simulink model "sschdlexVoltageSourceInverterModel"  (R2026a)
settings: Solver=FixedStepDiscrete  StopTime=0.03
InitFcn:
  | ts = 1e-005;
undefined symbols (not defined in the file or in its folder): Down, Up
libraries: fl_lib x11, nesl_utility x11, ee_lib x6, simulink x3, eeGeneralControl x1
CloseFcn:
  | clear all;
settings Model: DataTypeOverride=Off  Creator=The MathWorks, Inc.  LastModifiedBy=The MathWorks, Inc.
settings OptimizationCC: ConditionallyExecuteInputs=off
settings DebuggingCC: AlgebraicLoopMsg=error  SingleTaskRateTransMsg=error
settings HardwareCC: ProdHWDeviceType=ASIC/FPGA->ASIC/FPGA  TargetBitPerLong=64.0  TargetBitPerPointer=64.0  TargetBitPerSizeT=64.0  TargetBitPerPtrDiffT=64.0  TargetLongLongMode=on  TargetIntDivRoundTo=Zero  TargetEndianess=LittleEndian  TargetWordSize=64.0  TargetHWDeviceType=Custom Processor->MATLAB Host Computer  ProdEqTarget=off
settings SimscapeCC: SimscapeNominalValues="[{\"value\":\"1\",\"unit\":\"A\"},{\"value\":\"1\",\"unit\":\"bar\"},{\"value\":\"1\",\"unit\":\"cm^2\"},{\"value\":\"1\",\"unit\":\"cm^3/s\"},{\"value\":\"1\",\"unit\":\"kJ/kg\"},{\"value\":\"1\",\"unit\":\"kW\"},{\"value\":\"1\",\"unit\":\"l\"},{\"value\":\"1\",\"unit\":\"N\"},{\"value\":\"1\",\"unit\":\"N*m\"},{\"value\":\"1\",\"unit\":\"V\"}]"  SimscapeLogType=none  SimscapeLogDataHistory=5000.0

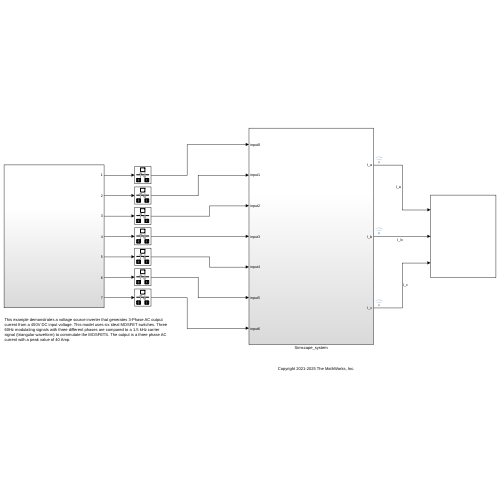
[thumbnail: Simulink's stored preview of the top-level diagram]
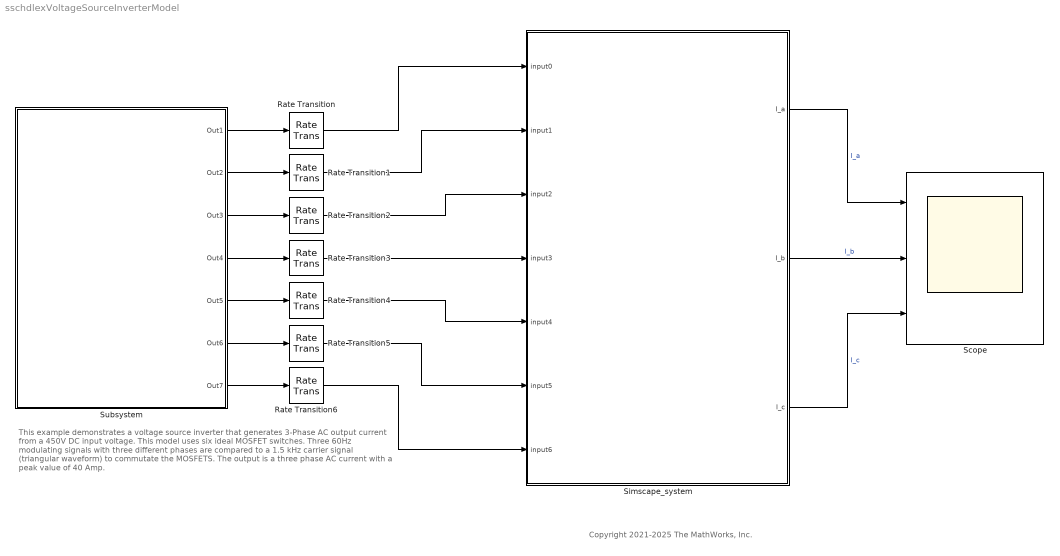
== system sschdlexVoltageSourceInverterModel ==
  note: This example demonstrates a voltage source inverter that generates 3-Phase AC output current from a 450V DC input voltage. This model uses six ideal MOSFET switches. Three 60Hz modulating signals with three different phases are compared to a 1.5 kHz carrier signal (triangular waveform) to commutate the MOSFETS. The output is a three phase AC current with a peak value of 40 Amp.
  note: Copyright 2021-2025 The MathWorks, Inc.
  Rate Transition{,1..6} (7 alike) : RateTransition
  Scope : Scope  NumInputPorts=3
      settings: ActiveDisplayYMinimum=-48.27085  ActiveDisplayYMaximum=49.00639
  Simscape_system : Subsystem
  Subsystem : Subsystem
  wires:
  Subsystem/1(Out1) -> Rate Transition/1
  Subsystem/7(Out7) -> Rate Transition6/1
  Subsystem/6(Out6) -> Rate Transition5/1
  Subsystem/5(Out5) -> Rate Transition4/1
  Subsystem/4(Out4) -> Rate Transition3/1
  Subsystem/3(Out3) -> Rate Transition2/1
  Subsystem/2(Out2) -> Rate Transition1/1
  Rate Transition/1 -> Simscape_system/1(input0)
  Rate Transition1/1 -> Simscape_system/2(input1)
  Rate Transition2/1 -> Simscape_system/3(input2)
  Rate Transition3/1 -> Simscape_system/4(input3)
  Rate Transition4/1 -> Simscape_system/5(input4)
  Rate Transition5/1 -> Simscape_system/6(input5)
  Rate Transition6/1 -> Simscape_system/7(input6)
  Simscape_system/2(I_b) -> Scope/2  "I_b"
  Simscape_system/1(I_a) -> Scope/1  "I_a"
  Simscape_system/3(I_c) -> Scope/3  "I_c"

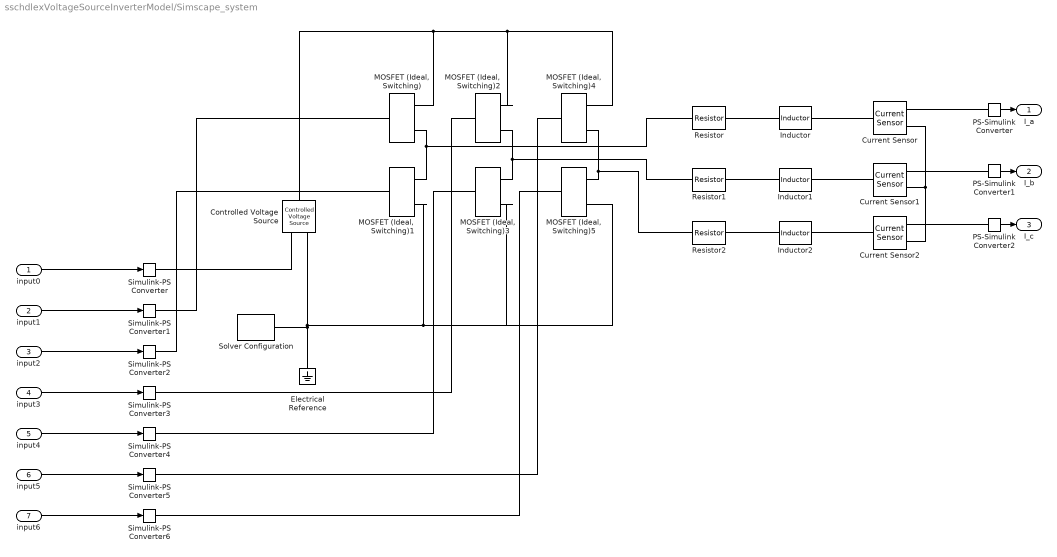
== system sschdlexVoltageSourceInverterModel/Simscape_system ==
  input0 : Inport
  input1 : Inport  Port=2
  input2 : Inport  Port=3
  input3 : Inport  Port=4
  input4 : Inport  Port=5
  input5 : Inport  Port=6
  input6 : Inport  Port=7
  Controlled Voltage Source : fl_lib/Electrical/Electrical Sources/Controlled Voltage Source
  Current Sensor : fl_lib/Electrical/Electrical Sensors/Current Sensor
  Current Sensor1 : fl_lib/Electrical/Electrical Sensors/Current Sensor
  Current Sensor2 : fl_lib/Electrical/Electrical Sensors/Current Sensor
  Electrical Reference : fl_lib/Electrical/Electrical Elements/Electrical Reference
  Inductor : fl_lib/Electrical/Electrical Elements/Inductor  l=0.0077 H  r=0 Ohm  g=1e-9 1/Ohm  i_specify=off  i_priority=None  i=0 A  i_nominal_specify=off  i_nominal_value=1  i_nominal_unit=A  v_specify=off  v_priority=None  v=0 V  v_nominal_specify=off  v_nominal_value=1  v_nominal_unit=V  i_L_specify=off  i_L_priority=High  i_L=0 A  i_L_nominal_specify=off  i_L_nominal_value=1  i_L_nominal_unit=A
  Inductor1 : fl_lib/Electrical/Electrical Elements/Inductor  l=0.0077 H  r=0 Ohm  g=1e-9 1/Ohm  i_specify=off  i_priority=None  i=0 A  i_nominal_specify=off  i_nominal_value=1  i_nominal_unit=A  v_specify=off  v_priority=None  v=0 V  v_nominal_specify=off  v_nominal_value=1  v_nominal_unit=V  i_L_specify=off  i_L_priority=High  i_L=0 A  i_L_nominal_specify=off  i_L_nominal_value=1  i_L_nominal_unit=A
  Inductor2 : fl_lib/Electrical/Electrical Elements/Inductor  l=0.0077 H  r=0 Ohm  g=1e-9 1/Ohm  i_specify=off  i_priority=None  i=0 A  i_nominal_specify=off  i_nominal_value=1  i_nominal_unit=A  v_specify=off  v_priority=None  v=0 V  v_nominal_specify=off  v_nominal_value=1  v_nominal_unit=V  i_L_specify=off  i_L_priority=High  i_L=0 A  i_L_nominal_specify=off  i_L_nominal_value=1  i_L_nominal_unit=A
  MOSFET (Ideal, Switching){,1..5} (6 alike) : ee_lib/Semiconductors & Converters/MOSFET (Ideal, Switching)  port_option=ee.enum.controlport.ps  Rds=0.001 Ohm  Goff=1e-6 1/Ohm  Vth=0.5 V  diode_param=2  diode_Vf=0.8 V  diode_Ron=0.001 Ohm  diode_Goff=1e-5 1/Ohm  diode_C=50e-9 F  diode_iRM=-235 A  diode_iF=300 A  diode_idot=-50 A/us  diode_trr_param=1  diode_trr_factor=3  diode_trr=15 us  diode_Qrr=1500 s*uA  ids_specify=off  ids_priority=None  ids=0 A  ids_nominal_specify=off  ids_nominal_value=1  ids_nominal_unit=A  vds_specify=off  vds_priority=None  vds=0 V  vds_nominal_specify=off  vds_nominal_value=1  vds_nominal_unit=V  vgs_specify=off  vgs_priority=None  vgs=0 V  vgs_nominal_specify=off  vgs_nominal_value=1  vgs_nominal_unit=V  thermal_loss_option=ee.enum.converters.thermalLossOption.constantvalues  Von_data=[0, 1.8, 3.2, 6, 10, 16; 0, 2, 5.5, 9.5, 15, 25] V  Tj=[298.15, 448.15] K  Iout_data=[0, 20, 40, 60, 80, 100] A  tabulateWithVds=false  Eon_data=[0, 55.04, 124.57, 235.53, 362.12; 0, 71.25, 161.25, 304.88, 468.75] * 1e-6 J  Eoff_data=[0, 18, 30, 56.1, 76.5; 0, 22.5, 37.5, 70.13, 95.63] * 1e-6 J  Eon_data_3D=[zeros(2, 5, 3)] J  Eoff_data_3D=[zeros(2, 5, 3)] J  Tj_loss=[298.15, 448.15] K  Iout_data_loss=[0, 10, 20, 30, 40] A  Vds_loss=[0, 150, 300] V  Eon_scalar=22.86e-3 J  Eoff_scalar=17.14e-3 J  Voff=300 V  Iout_scalar=600 A  useCurrentFromPreviousCycle=false  useVoltageFromPreviousCycle=false  diodeModelType=ee.enum.converters.diodeModelType.pwl  diodeTableType=ee.enum.diode.tableType.IfMat  diode_ReverseIVType=ee.enum.diode.diodeReverseIV.constant  diode_IfMat=[.07, .12, .19, 1.75, 4.24, 7.32, 11.2; .16, .3, .72, 2.14, 4.02, 6.35, 9.12] A  diode_VfMat=[.9, 1.15, 1.25, 1.5, 1.75, 2.17, 2.6, 2.85; .58, .68, .75, 1.1, 1.38, 1.77, 2.27, 2.7] V  diode_TjVec=[25, 125] degC  diode_VfVec=[.5, .7, .9, 1.3, 1.7, 2.1, 2.5] V  diode_IfVec=[.1, .2, .5, 1, 2, 4, 7, 10] A  diode_IrMat=[1e-06, 2e-06, 5e-06, 1e-05, 2.5e-05, 5e-05, .0001; 2e-06, 5e-06, 1e-05, 4e-05, 8e-05, .0002, .0005] A  diode_VrMat=[10, 100, 200, 250, 300, 325, 350; 10, 70, 160, 220, 270, 300, 320] V  diode_VrVec=[10, 20, 40, 50, 70, 80, 100] V  diode_IrVec=[1e-06, 2e-06, 5e-06, 1e-05, 2e-05, 5e-05, .0001] A  diode_Vr=-600 V  diode_Ls=150 nH  diode_Erec=0.03 J  diode_rec_loss_model=ee.enum.diode.reverseRecoveryModel.fixed  diode_ErecVal=0 J  diode_scaleWithIandV=true  diode_ErecMat=zeros(2, 3) J  diodeErecMat3D=zeros(2, 3, 2) J  diode_TjrecVec=[298.15, 398.15] K  diode_IfrecVec=[.1, 1, 10] A  diodeVrecVec=[0, 100] V  diode_IrecVal=10 A  diode_VrecVal=10 V  diode_tFilter=1 / 1000 / 100 s  separateThermalPortForDiode=false  thermal_network_parameterization=ee.enum.thermalNetworkTopology.external  Rth=[.03, .2] K/W  Rth_Cauer=[.03, .1, .2] K/W  Rth_Foster=[.03, .2] K/W  thermal_mass_parameterization=ee.enum.thermalNetwork.timeconstant  thermal_mass=[3, 25] J/K  thermal_mass_Cauer=[3, 10, 25] J/K  thermal_mass_Foster=[33, 50] J/K  thermal_time_constant=[.1, 5] s  thermal_time_constant_Cauer=[.1, 1, 5] s  thermal_time_constant_Foster=[1, 10] s  thermal_mass_initial_temperatures=[25, 25] degC  thermal_mass_initial_temperatures_Cauer=[25, 25, 25] degC  junction_thermal_mass=0.1 J/K  Tvec_initial_Foster=[25, 25, 25, 25] degC  RthDiode=[.03, .2] K/W  RthCauerDiode=[.03, .1, .2] K/W  RthFosterDiode=[.03, .2] K/W  thermalMassDiode=[3, 25] J/K  thermalMassCauerDiode=[3, 10, 25] J/K  thermalMassFosterDiode=[33, 50] J/K  thermalTauDiode=[.1, 5] s  thermalTauCauerDiode=[.1, 1, 5] s  thermalTauFosterDiode=[1, 10] s  thermalMassInitTempDiode=[25, 25] degC  thermalMassInitTempCauerDiode=[25, 25, 25] degC  junctionthermalMassDiode=0.1 J/K  TVecInitialFosterDiode=[25, 25, 25, 25] degC  no_thermal_network=0  mosfet_junction_temperature_specify=off  mosfet_junction_temperature_priority=None  mosfet_junction_temperature=25 degC  mosfet_junction_temperature_nominal_specify=off  mosfet_junction_temperature_nominal_value=1  mosfet_junction_temperature_nominal_unit=degC  diode_junction_temperature_specify=off  diode_junction_temperature_priority=None  diode_junction_temperature=25 degC  diode_junction_temperature_nominal_specify=off  diode_junction_temperature_nominal_value=1  diode_junction_temperature_nominal_unit=degC  Qj_specify=off  Qj_priority=None  Qj=0 W  Qj_nominal_specify=off  Qj_nominal_value=1  Qj_nominal_unit=W  accumulatedSwitchingLosses_specify=off  accumulatedSwitchingLosses_priority=None  accumulatedSwitchingLosses=0 J
  PS-Simulink Converter : nesl_utility/PS-Simulink Converter  PhysicalDomain=network_engine_domain  SubClassName=ps_output  LeftPortType=input  RightPortType=output  PseudoPeriodic=off  Frequencies=[]  VectorFormat=1-D array  Unit=inherit  AffineConversion=off
  PS-Simulink Converter1 : nesl_utility/PS-Simulink Converter  PhysicalDomain=network_engine_domain  SubClassName=ps_output  LeftPortType=input  RightPortType=output  PseudoPeriodic=off  Frequencies=[]  VectorFormat=1-D array  Unit=inherit  AffineConversion=off
  PS-Simulink Converter2 : nesl_utility/PS-Simulink Converter  PhysicalDomain=network_engine_domain  SubClassName=ps_output  LeftPortType=input  RightPortType=output  PseudoPeriodic=off  Frequencies=[]  VectorFormat=1-D array  Unit=inherit  AffineConversion=off
  Resistor : fl_lib/Electrical/Electrical Elements/Resistor  R=3.87 Ohm  i_specify=off  i_priority=None  i=0 A  i_nominal_specify=off  i_nominal_value=1  i_nominal_unit=A  v_specify=off  v_priority=None  v=0 V  v_nominal_specify=off  v_nominal_value=1  v_nominal_unit=V
  Resistor1 : fl_lib/Electrical/Electrical Elements/Resistor  R=3.87 Ohm  i_specify=off  i_priority=None  i=0 A  i_nominal_specify=off  i_nominal_value=1  i_nominal_unit=A  v_specify=off  v_priority=None  v=0 V  v_nominal_specify=off  v_nominal_value=1  v_nominal_unit=V
  Resistor2 : fl_lib/Electrical/Electrical Elements/Resistor  R=3.87 Ohm  i_specify=off  i_priority=None  i=0 A  i_nominal_specify=off  i_nominal_value=1  i_nominal_unit=A  v_specify=off  v_priority=None  v=0 V  v_nominal_specify=off  v_nominal_value=1  v_nominal_unit=V
  Simulink-PS Converter{,1..6} (7 alike) : nesl_utility/Simulink-PS Converter  PhysicalDomain=network_engine_domain  SubClassName=ps_input  LeftPortType=input  RightPortType=output  PseudoPeriodic=off  Frequencies=[]  NoiseDistribution=none  NoiseParameters=[]  Unit=1  AffineConversion=off  FilteringAndDerivatives=provide  SimscapeFilterOrder=1  InputFilterTimeConstant=0.001  UdotUserProvided=0
  Solver Configuration : nesl_utility/Solver Configuration  PhysicalDomain=network_engine_domain  SubClassName=solver  LeftPortType=input  RightPortType=generic  Tones=[]  Harmonics=[]  SimulateNoise=off  Profile=off  UseLocalSampling=off  EnableSwitchedLinearOptims=on  FrequencyDomain=off  UseCCode=off  RelTol=0.001  AbsTol=1e-06  MinStep=1e-09  ToWorkspace=off  RevertToSquareIcSolve=off  NumHomotopyIterations=100  PhasorMode=off  PhasorModeNumHarmonics=1  ConsistencySolver=NEWTON_FTOL  CanonicalOrdering=UNORDERED  OptimizeIntermediates=UNOPTIMIZED  IndexReductionMethod=DerivativeReplacement  DoDC=off  ResidualTolerance=1e-09  ConsistencyTolSource=GLOBAL  ConsistencyAbsTol=0.001  ConsistencyRelTol=0.001  ConsistencyTolFactor=0.001  UseLocalSolver=on  LocalSolverChoice=NE_BACKWARD_EULER_ADVANCER  ResolveIndetEquations=on  FunctionEvalNumThread=1  LocalSolverSampleTime=ts  DoFixedCost=off  MaxNonlinIter=1  MaxModeIter=2  ComputeImpulses=off  ImpulseIterations=1  LinearAlgebra=auto  LinearAlgebraNumThread=0  EquationFormulation=NE_TIME_EF  DelaysMemoryBudget=1024  AutomaticFiltering=on  FilteringTimeConstant=0.001  PartitionStorageMethod=AS_NEEDED  PartitionMemoryBudget=1024  PartitionMethod=ROBUST  MultibodyUseLocalSolver=off  MultibodyLocalSolverChoice=ODE1  MultibodyLocalSolverSampleTime=0.001
  I_a : Outport
  I_b : Outport  Port=2
  I_c : Outport  Port=3
  wires:
  PS-Simulink Converter2/1 -> I_c/1
  input6/1 -> Simulink-PS Converter6/1
  input2/1 -> Simulink-PS Converter2/1
  input4/1 -> Simulink-PS Converter4/1
  input5/1 -> Simulink-PS Converter5/1
  PS-Simulink Converter/1 -> I_a/1
  input3/1 -> Simulink-PS Converter3/1
  input1/1 -> Simulink-PS Converter1/1
  input0/1 -> Simulink-PS Converter/1
  PS-Simulink Converter1/1 -> I_b/1
  connections:
  Simulink-PS Converter5/RConn1 -- "MOSFET (Ideal, Switching)4"/LConn1
  Simulink-PS Converter2/RConn1 -- "MOSFET (Ideal, Switching)1"/LConn1
  Inductor1/LConn1 -- Resistor1/RConn1
  PS-Simulink Converter/LConn1 -- Current Sensor/RConn1
  Current Sensor2/LConn1 -- Inductor2/RConn1
  "MOSFET (Ideal, Switching)2"/RConn2 -- Resistor1/LConn1 -- "MOSFET (Ideal, Switching)3"/RConn1
  Inductor/LConn1 -- Resistor/RConn1
  PS-Simulink Converter2/LConn1 -- Current Sensor2/RConn1
  PS-Simulink Converter1/LConn1 -- Current Sensor1/RConn1
  "MOSFET (Ideal, Switching)4"/RConn1 -- "MOSFET (Ideal, Switching)2"/RConn1 -- Controlled Voltage Source/LConn1 -- "MOSFET (Ideal, Switching)"/RConn1
  Simulink-PS Converter3/RConn1 -- "MOSFET (Ideal, Switching)2"/LConn1
  Simulink-PS Converter/RConn1 -- Controlled Voltage Source/RConn1
  Inductor2/LConn1 -- Resistor2/RConn1
  Simulink-PS Converter6/RConn1 -- "MOSFET (Ideal, Switching)5"/LConn1
  Electrical Reference/LConn1 -- "MOSFET (Ideal, Switching)3"/RConn2 -- "MOSFET (Ideal, Switching)5"/RConn2 -- "MOSFET (Ideal, Switching)1"/RConn2 -- Controlled Voltage Source/RConn2 -- Solver Configuration/RConn1
  Current Sensor/LConn1 -- Inductor/RConn1
  "MOSFET (Ideal, Switching)4"/RConn2 -- "MOSFET (Ideal, Switching)5"/RConn1 -- Resistor2/LConn1
  Current Sensor/RConn2 -- Current Sensor1/RConn2 -- Current Sensor2/RConn2
  "MOSFET (Ideal, Switching)"/RConn2 -- Resistor/LConn1 -- "MOSFET (Ideal, Switching)1"/RConn1
  Current Sensor1/LConn1 -- Inductor1/RConn1
  Simulink-PS Converter4/RConn1 -- "MOSFET (Ideal, Switching)3"/LConn1
  Simulink-PS Converter1/RConn1 -- "MOSFET (Ideal, Switching)"/LConn1

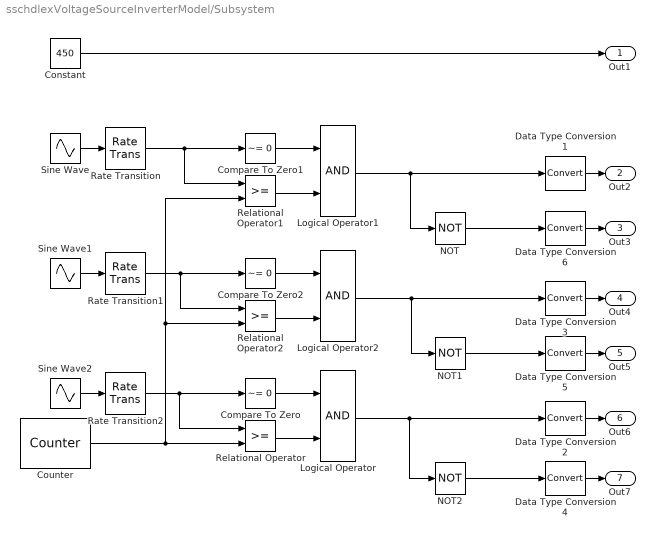
== system sschdlexVoltageSourceInverterModel/Subsystem ==
  Compare To Zero : simulink/Logic and Bit Operations/Compare To Zero  relop=~=  OutDataTypeStr=boolean
  Compare To Zero1 : simulink/Logic and Bit Operations/Compare To Zero  relop=~=  OutDataTypeStr=boolean
  Compare To Zero2 : simulink/Logic and Bit Operations/Compare To Zero  relop=~=  OutDataTypeStr=boolean
  Constant : Constant  Value=450  SampleTime=-1
  Counter : eeGeneralControl/Counter  CarrCount=Up-Down  Range=[-1 1]  Tper=1/(2*1.5e3)  Tdelay=0  Ts=ts/3
      settings: LibrarySourceBlock=ee_sl_lib/General Control/Counter
  Data Type Conversion{1..6} (6 alike) : DataTypeConversion  SaturateOnIntegerOverflow=off  RndMeth=Floor
  Logical Operator : Logic  AllPortsSameDT=off  OutDataTypeStr=boolean
  Logical Operator1 : Logic  AllPortsSameDT=off  OutDataTypeStr=boolean
  Logical Operator2 : Logic  AllPortsSameDT=off  OutDataTypeStr=boolean
  NOT : Logic  Operator=NOT  IconShape=distinctive  AllPortsSameDT=off  OutDataTypeStr=boolean
  NOT1 : Logic  Operator=NOT  IconShape=distinctive  AllPortsSameDT=off  OutDataTypeStr=boolean
  NOT2 : Logic  Operator=NOT  IconShape=distinctive  AllPortsSameDT=off  OutDataTypeStr=boolean
  Rate Transition : RateTransition
  Rate Transition1 : RateTransition
  Rate Transition2 : RateTransition
  Relational Operator : RelationalOperator  OutDataTypeStr=boolean  RndMeth=Simplest  InputSameDT=off
  Relational Operator1 : RelationalOperator  OutDataTypeStr=boolean  RndMeth=Simplest  InputSameDT=off
  Relational Operator2 : RelationalOperator  OutDataTypeStr=boolean  RndMeth=Simplest  InputSameDT=off
  Sine Wave : Sin  Amplitude=0.8  Frequency=2 * pi * 60  SampleTime=0
  Sine Wave1 : Sin  Amplitude=0.8  Frequency=2 * pi * 60  Phase=-120 * pi/180  SampleTime=0
  Sine Wave2 : Sin  Amplitude=0.8  Frequency=2 * pi * 60  Phase=-240 * pi/180  SampleTime=0
  Out1 : Outport
  Out2 : Outport  Port=2
  Out3 : Outport  Port=3
  Out4 : Outport  Port=4
  Out5 : Outport  Port=5
  Out6 : Outport  Port=6
  Out7 : Outport  Port=7
  wires:
  Compare To Zero/1 -> Logical Operator/1
  Data Type Conversion4/1 -> Out7/1
  NOT2/1 -> Data Type Conversion4/1
  Compare To Zero1/1 -> Logical Operator1/1
  NOT/1 -> Data Type Conversion6/1
  Relational Operator/1 -> Logical Operator/2
  Logical Operator1/1 -> NOT/1, Data Type Conversion1/1
  NOT1/1 -> Data Type Conversion5/1
  Data Type Conversion1/1 -> Out2/1
  Sine Wave1/1 -> Rate Transition1/1
  Relational Operator1/1 -> Logical Operator1/2
  Sine Wave/1 -> Rate Transition/1
  Data Type Conversion5/1 -> Out5/1
  Logical Operator/1 -> NOT2/1, Data Type Conversion2/1
  Logical Operator2/1 -> Data Type Conversion3/1, NOT1/1
  Compare To Zero2/1 -> Logical Operator2/1
  Constant/1 -> Out1/1
  Relational Operator2/1 -> Logical Operator2/2
  Data Type Conversion3/1 -> Out4/1
  Data Type Conversion2/1 -> Out6/1
  Sine Wave2/1 -> Rate Transition2/1
  Data Type Conversion6/1 -> Out3/1
  Counter/1 -> Relational Operator/2, Relational Operator2/2, Relational Operator1/2
  Rate Transition/1 -> Relational Operator1/1, Compare To Zero1/1
  Rate Transition1/1 -> Compare To Zero2/1, Relational Operator2/1
  Rate Transition2/1 -> Compare To Zero/1, Relational Operator/1
